simulink model "SMART_DC_CHARGING_MODEL"  (R2026b)
settings: Solver=VariableStepAuto
settings Model: Creator=HP  LastModifiedBy=HP

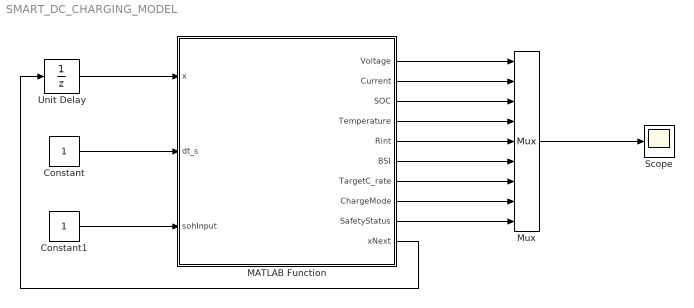
== system SMART_DC_CHARGING_MODEL ==
  Constant : Constant
  Constant1 : Constant
  MATLAB Function : MATLAB Function  TreatAsAtomicUnit=on
  Mux : Mux  Inputs=9
  Scope : Scope
      settings: ActiveDisplayYMinimum=-3.1265372492694947  ActiveDisplayYMaximum=28.138835243425461
  Unit Delay : UnitDelay  InitialCondition=[0.20;25;0;1]  SampleTime=-1
  wires:
  Unit Delay/1 -> MATLAB Function/1(x)
  Constant1/1 -> MATLAB Function/3(sohInput)
  Constant/1 -> MATLAB Function/2(dt_s)
  MATLAB Function/10(xNext) -> Unit Delay/1
  MATLAB Function/1(Voltage) -> Mux/1
  MATLAB Function/2(Current) -> Mux/2
  MATLAB Function/3(SOC) -> Mux/3
  MATLAB Function/4(Temperature) -> Mux/4
  MATLAB Function/5(Rint) -> Mux/5
  MATLAB Function/6(BSI) -> Mux/6
  MATLAB Function/7(TargetC_rate) -> Mux/7
  MATLAB Function/8(ChargeMode) -> Mux/8
  MATLAB Function/9(SafetyStatus) -> Mux/9
  Mux/1 -> Scope/1

== matlab function SMART_DC_CHARGING_MODEL/MATLAB Function ==
  data: x input double size=[4, 1]; Voltage output; dt_s input; sohInput input; Current output; SOC output; Temperature output; Rint output; BSI output; TargetC_rate output; ChargeMode output; SafetyStatus output; xNext output double size=[4, 1]
function [Voltage, Current, SOC, Temperature, Rint, BSI, TargetC_rate, ChargeMode, SafetyStatus, xNext] = smart_battery_model(x, dt_s, sohInput)
